simulink model "sf_battery_management"  (R2025b)
settings: Solver=FixedStepAuto  StartTime=0.0  StopTime=inf  FixedStep=0.1  RelTol=1e-3
PreLoadFcn:
  | load('battery_management_data.mat')
values from neighbouring files (symbols this model uses):
  CODEGEN_FLAG = 0    [battery_management_data.mat]
  currentFaultSim = 0    [battery_management_data.mat]
  currentSensorSim = 0    [battery_management_data.mat]
  tempFaultSim = 0    [battery_management_data.mat]
  tempSensorSim = 0    [battery_management_data.mat]
  voltageFaultSim = 0    [battery_management_data.mat]
  voltageSensorSim = 0    [battery_management_data.mat]
(part 2 of 3)

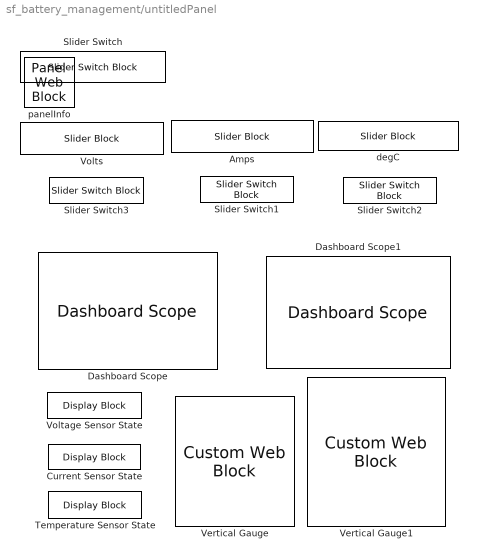
== system sf_battery_management/untitledPanel ==
  Amps : SliderBlock  Tag=HiddenForWebPanel  PanelInfo="{\"height\":32,\"left\":162,\"panelId\":\"panelId-91335c16-9517-4c37-953d-f6a6e757ae52\",\"top\":78,\"type\":\"panelChild\",\"version\":\"2019b\",\"width\":142,\"zIndex\":2000844}"  LabelPosition=Hide  ScaleMax=500  TickInterval=125
  Current Sensor State : DisplayBlock  Tag=HiddenForWebPanel  PanelInfo="{\"height\":25,\"left\":39,\"panelId\":\"panelId-91335c16-9517-4c37-953d-f6a6e757ae52\",\"top\":402,\"type\":\"panelChild\",\"version\":\"2019b\",\"width\":92,\"zIndex\":1500016}"  LabelPosition=Hide  Transparency=1  GridColor=[0.502, 0.502, 0.502]
  Dashboard Scope : DashboardScope  Tag=HiddenForWebPanel  PanelInfo="{\"height\":117,\"left\":29,\"panelId\":\"panelId-91335c16-9517-4c37-953d-f6a6e757ae52\",\"top\":210,\"type\":\"panelChild\",\"version\":\"2019b\",\"width\":179,\"zIndex\":2000856}"  TimeSpan=10  Ymin=100  Ymax=300  LegendPosition=Hide  ScaleAtStop=off  FontColor=[0.0, 0.0, 0.0]
  Dashboard Scope1 : DashboardScope  Tag=HiddenForWebPanel  PanelInfo="{\"height\":112,\"left\":257,\"panelId\":\"panelId-91335c16-9517-4c37-953d-f6a6e757ae52\",\"top\":214,\"type\":\"panelChild\",\"version\":\"2019b\",\"width\":184,\"zIndex\":2000858}"  TimeSpan=10  Ymin=0  Ymax=100  LegendPosition=Hide  ScaleAtStop=off  FontColor=[0.0, 0.0, 0.0]
  Slider Switch : SliderSwitchBlock  Tag=HiddenForWebPanel  PanelInfo="{\"height\":31,\"left\":11,\"panelId\":\"panelId-91335c16-9517-4c37-953d-f6a6e757ae52\",\"top\":9,\"type\":\"panelChild\",\"version\":\"2019b\",\"width\":145,\"zIndex\":2000854}"  LabelPosition=Hide
  Slider Switch1 : SliderSwitchBlock  Tag=HiddenForWebPanel  PanelInfo="{\"height\":26,\"left\":191,\"panelId\":\"panelId-91335c16-9517-4c37-953d-f6a6e757ae52\",\"top\":134,\"type\":\"panelChild\",\"version\":\"2019b\",\"width\":93,\"zIndex\":2000862}"  LabelPosition=Hide
  Slider Switch2 : SliderSwitchBlock  Tag=HiddenForWebPanel  PanelInfo="{\"height\":26,\"left\":334,\"panelId\":\"panelId-91335c16-9517-4c37-953d-f6a6e757ae52\",\"top\":135,\"type\":\"panelChild\",\"version\":\"2019b\",\"width\":93,\"zIndex\":2000864}"  LabelPosition=Hide
  Slider Switch3 : SliderSwitchBlock  Tag=HiddenForWebPanel  PanelInfo="{\"height\":26,\"left\":40,\"panelId\":\"panelId-91335c16-9517-4c37-953d-f6a6e757ae52\",\"top\":135,\"type\":\"panelChild\",\"version\":\"2019b\",\"width\":94,\"zIndex\":2000860}"  LabelPosition=Hide
  Temperature Sensor State : DisplayBlock  Tag=HiddenForWebPanel  PanelInfo="{\"height\":27,\"left\":39,\"panelId\":\"panelId-91335c16-9517-4c37-953d-f6a6e757ae52\",\"top\":449,\"type\":\"panelChild\",\"version\":\"2019b\",\"width\":93,\"zIndex\":1500014}"  LabelPosition=Hide  Transparency=1  GridColor=[0.502, 0.502, 0.502]
  Vertical Gauge : CustomWebBlock  Tag=HiddenForWebPanel  PanelInfo="{\"height\":130,\"left\":166,\"panelId\":\"panelId-91335c16-9517-4c37-953d-f6a6e757ae52\",\"top\":354,\"type\":\"panelChild\",\"version\":\"2019b\",\"width\":119,\"zIndex\":1500008}"  LabelPosition=Hide  ShowInitialText=on  Configuration="{\"components\":[{\"name\":\"LinearScaleComponent\",\"settings\":{\"bounds\":{\"max\":4.5,\"min\":-0.5,\"tickInterval\":1},\"labelColor\":[0,85,255],\"labelFont\":{\"font\":\"Arial\",\"fontSize\":12},\"labelOffset\":0.05,\"labelTransparency\":0,\"needleImage\":{\"size\":[109,53],\"src\":\"data:image\\/png;base64,iVBORw0KGgoAAAANSUhEUgAAAG0AAAA1CAMAAAB8+5X+AAAAAXNSR0IArs4c6QAAAARnQU1BAACxjwv8YQUAAAByUExURQAAAP8AAP8AAP8AAP8AAP8AAP8AAP8AAP8AAP8AAP8AAP8AAP8AAP8AAP8AAP8AAP8AAP8AAP8AAP8AAP8AAP8AAP8AAP8AAP8AAP8AAP8AAP8AAP8AAP8AAP8AAP8AAP8AAP8AAP8AAP8AAP8AAP8AAImxNnoAAAAldFJOUwAEDBAUGBwgJDQ4PFBUWHR4fICTl5ufo6+zt7u\\/w8\\/T1+fz9\\/snRUfzAAAACXBIWXMAABcRAAAXEQHKJvM\\/AAABCUlEQVRYR92Yxw7CQAxEQ++99ySw\\/\\/+LlDyJAAsnew68E9iWRxFDdu0kmDKrJD+hzIpNlb5xqDLj2KBxFIrsyDp0jkGNIXmf1hEoseQyovcnVNgy\\/2ZN8sZsv1iTtDWnJv1fIWtO3Jok7ckHKJQh58EYiRJkXFh8WJOED7t3axJ3Im0hA4S9yLroFBB1Ix8i9ICgIxOU7hDyZPm0JhFX9jXEJGohbSvVQtZTqoVzYU2++TOVqoXVzZp8VHCoK9XC+m+fTfq7KT0p\\/b9J3yXS96T0DJCeb8qzW3ovkd65pPdJ6V1ZOgcoZxzp\\/CadTaVzt3SnoNyXSHdB0j2XdIcn3U9Kd68\\/98pJcgVZGsxjzJl\\/4AAAAABJRU5ErkJggg==\",\"srcOrientation\":\"Right\"},\"needleOffset\":[-0.0013831258644536654,-0.18488023952095808],\"needleSize\":{\"height\":0.07432154605263158,\"width\":0.1941860465116279},\"position\":[0.2313939144736842,0.12056686046511628,0.41540697674418603,0.6739823190789473],\"referencePoint\":\"auto\",\"scaleColorSize\":0.24,\"scaleColors\":[],\"scaleColorsSize\":0.2,\"scaleDirection\":\"BT\",\"tickColor\":[0,0,0],\"tickTransparency\":0.8,\"valueBarColor\":[81,255,0],\"valueBarSize\":0.23,\"valueBarTransparency\":1}},{\"name\":\"BackgroundImageComponent\",\"settings\":{\"image\":{\"size\":[776,978],\"src\":\"data:image\\/png;base64,iVBORw0KGgoAAAANSUhEUgAAAwgAAAPSCAYAAADfoP1eAAAAAXNSR0IArs4c6QAAAARnQU1BAACxjwv8YQUAAAAJcEhZcwAAFxEAABcRAcom8z8AAN6TSURBVHhe7P1ZuB1Xde\\/9\\/y\\/OxXtxLs7FuTgX53ne9+I8cSsJAgSSkNCEA4TWsiEhIaFJSEhHQughELoAobFkg8GAgzEY95ZkNZas3pYty5Z7tVbfd1bf91r\\/Gku15a2t315zzlpzrVVjr+\\/g+TyAvWtWrbn3nDXGqqpZ\\/z\\/Cf1x97Q8uH33NDe8ac+34jzSNHf+1pmvH3zx67LhfFv99X\\/Hf88dcO+7R0deO22CKf3+8+OcNAADgw+hrx5++cB63c3pxbi9MKs ...(+78488 chars)\",\"srcOrientation\":\"vertical\"},\"position\":[0,0,1,1],\"scaleMode\":\"0\"}},{\"name\":\"ForegroundImageComponent\",\"settings\":{\"image\":{\"size\":[0,0],\"src\":\"default\",\"srcOrientation\":\"\"},\"isForeground\":1,\"position\":[0,0,1,1]}}],\"derived\":{\"blockParameters\":{\"ForegroundColor\":[0,0,0],\"Limits\":{\"Max\":4.5,\"Min\":-0.5,\"Ticks\":1},\"ScaleColors\":[],\"ScaleDirection\":\"Clockwise\",\"ScaleMax\":4.5,\"ScaleMin\":-0.5,\"TickInterval\":1,\"fixedAspectRatio\":\"on\"}},\"settings\":{\"BindingType\":\"signal\",\"backgroundColor\":[0,0,0],\"backgroundOffset\":0,\"backgroundOpacity\":1,\"fixedAspectRatio\":\"on\",\"orientation\":\"vertical\",\"showBackgroundColor\":0,\"version\":\"R2025a\"},\"type\":\"LinearGauge\"}"
  Vertical Gauge1 : CustomWebBlock  Tag=HiddenForWebPanel  PanelInfo="{\"height\":149,\"left\":298,\"panelId\":\"panelId-91335c16-9517-4c37-953d-f6a6e757ae52\",\"top\":335,\"type\":\"panelChild\",\"version\":\"2019b\",\"width\":138,\"zIndex\":1500022}"  LabelPosition=Hide  ShowInitialText=on  Configuration="{\"components\":[{\"name\":\"LinearScaleComponent\",\"settings\":{\"bounds\":{\"max\":2.5,\"min\":-2.5,\"tickInterval\":1},\"labelColor\":[0,85,255],\"labelFont\":{\"font\":\"Arial\",\"fontSize\":12},\"labelOffset\":0.05,\"labelTransparency\":0,\"needleImage\":{\"size\":[80,81],\"src\":\"data:image\\/png;base64,iVBORw0KGgoAAAANSUhEUgAAAFAAAABRCAMAAAByk9E6AAAAAXNSR0IArs4c6QAAAARnQU1BAACxjwv8YQUAAADVUExURQAAAEBAgCBggDBQjytVii5SkjJVji1TjDBQjy9RkTBUjzBTjy5SjzBSjy5SjzBSjy5RjzBSjy9SjjBTjy5SjzBSjy9Sjy9Sjy9Tji9SkC9Rjy9Sjy5Sjy9Tjy9SkC9Sjy9Sjy9SkC9Sjy9Sjy9SkC9SjzBSkjBUky9Sjy9TkDBSkTBTkTBUkjFVlDJWlzNYmTRZmzRanDVbnjVcnzZdoTdeozhgpjlhqDpiqjpjqztkrTxmsD5otD9qt0BsukBsu0FuvEFuvUJvv0NwwUNxwkRxw0RyxLvf0MQAAAAodFJOUwAECBAYHCQoMDxAUFRgZHB0gIOLj5ufr7O3v8PLz9fb4+fr7\\/f7\\/v5uSHl1AAAACXBIWXMAABcRAAAXEQHKJvM\\/AAAB+0lEQVRYR63Y2VbCMBAG4Ir7voviioLGfQVRBJFl3v+RnNAUCm3TyWT+u\\/Yk3017JpMJ1mcC2ahzYVIpYVKpRyTXzJNAlOp\\/I3m6ap69oxSAKKlBUTIENfkgQ0YgQK+B5MmKec\\/OGDRkyZOMgyLkJChAToNIft77kEkQoFtH8nDJrHBMGqjJO6WKLDId9CCzQDaZDSJZu3UnbSBAB8nqwYJZS4odZJB5oDOZDzqSFBDg910hOW\\/2WEMDAdpIVvbmzC5LqCCZpINE0gUkkW4gQOsVyd1ZszslrmBIXm1nku5gDskBrSQPRPIlg+SCAD\\/PSG4VjDMKHwzJ8uYU6QOmkn5gCukLIvk0QfqDMGgieRH11QKgIU2rLgLGSSEQyQ+8UBwVxMDR15YBYz+PBKi5y+jH8QdbyMXKhC+YKGR+YEpd9AFTyywf1FxlJ1FiuWD7LeNA5YGW85kDWo97dzCne3AFNVfdtzQjbmCnpvtEa+vpApI6WTpIbIypILnPpoF\\/yKniotljDQXs1q\\/pN6p80InLBx25PJBxI7WBPc2Vls1KYrLBXuOGM3vIAplcFsjm0sHh7OaYOWhJgv0v5PhjtWnQe\\/A3CQrMEeOgyFhyDA65M++RZAQOmshJDKBDMN4ke0aDgpwGRTkNIlfekOI0OH1Z84wwFwSyXBD8AwOyKt7SV8XcAAAAAElFTkSuQmCC\",\"srcOrientation\":\"Right\"},\"needleOffset\":[-0.03305785123966942,-0.28908964558721334],\"needleSize\":{\"height\":0.1281779661016949,\"width\":0.08817401960784314},\"position\":[0.1421875,0.19939630681818182,0.2859552556818182,0.8486842105263158],\"referencePoint\":\"auto\",\"scaleColorSize\":0.24,\"scaleColors\":[],\"scaleColorsSize\":0.2,\"scaleDirection\":\"BT\",\"tickColor\":[0,0,0],\"tickTransparency\":0.9,\"valueBarColor\":[81,255,0],\"valueBarSize\":0.23,\"valueBarTransparency\":0}},{\"name\":\"BackgroundImageComponent\",\"settings\":{\"image\":{\"size\":[852,986],\"src\":\"data:image\\/png;base64,iVBORw0KGgoAAAANSUhEUgAAA1QAAAPaCAYAAACQ2xn1AAAAAXNSR0IArs4c6QAAAARnQU1BAACxjwv8YQUAAAAJcEhZcwAAFxEAABcRAcom8z8AAOWhSURBVHhe7P1rtDVnXed754UvfLGHyYt+0S\\/2EB3DwX1ed8IxQPAGEpIYCMm6E5SD4dwQWg42IRhAzAEldkjWCgpiGyGgtlE5oy0ICO7dqBt9xqPI2Nt2d6tt293SQ3sjjTY+0L3Xs35zrUrmXfldV9X\\/qqo5q2p+rzE+Su5Vp1lVs+b\\/V4erzqNtZjtz5tZvOXn27qOnr9t9yqntnetPn9190da1Ozee3t69beHs7ru3tnfu3\\/\\/\\/H9j\\/\\/59bOLvz54e+sv\\/vew ...(+80792 chars)\",\"srcOrientation\":\"vertical\"},\"position\":[0,0,1,1],\"scaleMode\":\"0\"}},{\"name\":\"ForegroundImageComponent\",\"settings\":{\"image\":{\"size\":[0,0],\"src\":\"default\",\"srcOrientation\":\"\"},\"isForeground\":1,\"position\":[0,0,1,1]}}],\"derived\":{\"blockParameters\":{\"ForegroundColor\":[0,0,0],\"Limits\":{\"Max\":2.5,\"Min\":-2.5,\"Ticks\":1},\"ScaleColors\":[],\"ScaleDirection\":\"Clockwise\",\"ScaleMax\":2.5,\"ScaleMin\":-2.5,\"TickInterval\":1,\"fixedAspectRatio\":\"on\"}},\"settings\":{\"BindingType\":\"signal\",\"backgroundColor\":[0,0,0],\"backgroundOffset\":0,\"backgroundOpacity\":1,\"fixedAspectRatio\":\"on\",\"orientation\":\"vertical\",\"showBackgroundColor\":0,\"version\":\"R2025a\"},\"type\":\"LinearGauge\"}"
  Voltage Sensor State : DisplayBlock  Tag=HiddenForWebPanel  PanelInfo="{\"height\":26,\"left\":38,\"panelId\":\"panelId-91335c16-9517-4c37-953d-f6a6e757ae52\",\"top\":350,\"type\":\"panelChild\",\"version\":\"2019b\",\"width\":94,\"zIndex\":1500018}"  LabelPosition=Hide  Transparency=1  GridColor=[0.502, 0.502, 0.502]
  Volts : SliderBlock  Tag=HiddenForWebPanel  PanelInfo="{\"height\":32,\"left\":11,\"panelId\":\"panelId-91335c16-9517-4c37-953d-f6a6e757ae52\",\"top\":80,\"type\":\"panelChild\",\"version\":\"2019b\",\"width\":143,\"zIndex\":2000842}"  LabelPosition=Hide  ScaleMin=100  ScaleMax=300  TickInterval=100
  degC : SliderBlock  Tag=HiddenForWebPanel  PanelInfo="{\"height\":29,\"left\":309,\"panelId\":\"panelId-91335c16-9517-4c37-953d-f6a6e757ae52\",\"top\":79,\"type\":\"panelChild\",\"version\":\"2019b\",\"width\":140,\"zIndex\":2000846}"  LabelPosition=Hide  ScaleMin=-50  ScaleMax=50  TickInterval=25
  panelInfo : PanelWebBlock  Tag=HiddenForWebPanel  PanelInfo="{\"compacted\":false,\"height\":496,\"isActiveTab\":true,\"labels\":{\"label0480254190\":{\"left\":\"244\",\"settings\":{\"backgroundColor\":\"rgba(0, 0, 0, 0)\",\"bold\":false,\"font\":\"Arial\",\"fontColor\":\"black\",\"fontSize\":0.71,\"italicized\":false,\"underlined\":false},\"text\":\"%\",\"top\":\"252\"},\"label1417532565\":{\"left\":\"170\",\"settings\":{\"backgroundColor\":\"rgba(0, 0, 0, 0)\",\"bold\":true,\"font\":\"Arial\",\"fontColor\":\"black\",\"fontSize\":0.86,\"italicized\":false,\"underlined\":false},\"text\":\"Signal Monitoring\",\"top\":\"172\"},\"label2677336777\":{\"left\":\"164\",\"settings\":{\"backgroundColor\":\"rgba(0, 0, 0, 0)\",\"bold\":true,\"font\":\"Arial\",\"fontColor\":\"black\",\"fontSize\":0.94,\"italicized\":false,\"underlined\":false},\"text\":\"State Monitoring\",\"top\":\"330\"},\"label3169608891\":{\"left\":\"70\",\"settings\":{\"backgroundColor\":\"rgba(0, 0, 0, 0)\",\"bold\":false,\"font\":\"Arial\",\"fontColor\":\"black\",\"fontSize\":0.71,\"italicized\":false,\"underlined\":false},\"text\":\"Voltage read from sensor\",\"top\":\"197\"},\"label4653890763\":{\"left\":\"56\",\"settings\":{\"backgroundColor\":\"rgba(0, 0, 0, 0)\",\"bold\":false,\"font\":\"Arial\",\"fontColor\":\"black\",\"fontSize\":0.71,\"italicized\":false,\"underlined\":false},\"text\":\"Voltage [V]\",\"top\":\"59\"},\"label5267384152\":{\"left\":\"319\",\"settings\":{\"backgroundColor\":\"rgba(0, 0, 0, 0)\",\"bold\":false,\"font\":\"Arial\",\"fontColor\":\"black\",\"fontSize\":0.55,\"italicized\":false,\"underlined\":false},\"text\":\"Send Temperature Error Code\",\"top\":\"123\"},\"label5437745661\":{\"left\":\"37\",\"settings\":{\"backgroundColor\":\"rgba(0, 0, 0, 0)\",\"bold\":false,\"font\":\"Arial\",\"fontColor\":\"black\",\"fontSize\":0.55,\"italicized\":false,\"underlined\":false},\"text\":\"Send Voltage Error Code\",\"top\":\"123\"},\"label6942438338\":{\"left\":\"331\",\"settings\":{\"backgroundColor\":\"rgba(0, 0, 0, 0)\",\"bold\":false,\"font\":\"Arial\",\"fontColor\":\"black\",\"fontSize\":0.71,\"italicized\":false,\"underlined\":false},\"text\":\"Temperature [degC]\",\"top\":\"57\"},\"label7286642277\":{\"left\":\"292\",\"settings\":{\"backgroundColor\":\"rgba(0, 0, 0, 0)\",\"bold\":false,\"font\":\"Arial\",\"fontColor\":\"black\",\"fontSize\":0.71,\"italicized\":false,\"underlined\":false},\"text\":\"SOC estimate from C code\",\"top\":\"199\"},\"label7883531891\":{\"left\":\"17\",\"settings\":{\"backgroundColor\":\"rgba(0, 0, 0, 0)\",\"bold\":false,\"font\":\"Arial\",\"fontColor\":\"black\",\"fontSize\":0.71,\"italicized\":false,\"underlined\":false},\"text\":\"Voltage Sensor Fault State\",\"top\":\"336\"},\"label8120698335\":{\"left\":\"205\",\"settings\":{\"backgroundColor\":\"rgba(0, 0, 0, 0)\",\"bold\":false,\"font\":\"Arial\",\"fontColor\":\"black\",\"fontSize\":0.71,\"italicized\":false,\"underlined\":false},\"text\":\"Current [A]\",\"top\":\"61\"},\"label8170647083\":{\"left\":\"9\",\"settings\":{\"backgroundColor\":\"rgba(0, 0, 0, 0)\",\"bold\":false,\"font\":\"Arial\",\"fontColor\":\"black\",\"fontSize\":0.71,\"italicized\":false,\"underlined\":false},\"text\":\"Volts\",\"top\":\"251\"},\"label8292420699\":{\"left\":\"9\",\"settings\":{\"backgroundColor\":\"rgba(0, 0, 0, 0)\",\"bold\":false,\"font\":\"Arial\",\"fontColor\":\"black\",\"fontSize\":0.71,\"italicized\":false,\"underlined\":false},\"text\":\"Temperature Sensor Fault State\",\"top\":\"436\"},\"label8302910947\":{\"left\":\"186\",\"settings\":{\"backgroundColor\":\"rgba(0, 0, 0, 0)\",\"bold\":true,\"font\":\"Arial\",\"fontColor\":\"black\",\"fontSize\":0.94,\"italicized\":false,\"underlined\":false},\"text\":\"Sensor Input\",\"top\":\"7\"},\"label8970115634\":{\"left\":\"18\",\"settings\":{\"backgroundColor\":\"rgba(0, 0, 0, 0)\",\"bold\":false,\"font\":\"Arial\",\"fontColor\":\"black\",\"fontSize\":0.71,\"italicized\":false,\"underlined\":false},\"text\":\"Current Sensor Fault State\",\"top\":\"387\"},\"label9336161722\":{\"left\":\"184\",\"settings\":{\"backgroundColor\":\"rgba(0, 0, 0, 0)\",\"bold\":false,\"font\":\"Arial\",\"fontColor\":\"black\",\"fontSize\":0.55,\"italicized\":false,\"underlined\":false},\"text\":\"Send Current Error Code\",\"top\":\"122\"}},\"left\":39,\"name\":\"untitledPanel\",\"panelId\":\"panelId-91335c16-9517-4c37-953d-f6a6e757ae52\",\"popoutData\":{\"height\":0,\"left\":0,\"maximized\":false,\"top\":0,\"width\":0},\"popoutMode\":\"component\",\"tabIndex\":0,\"tabbedSetId\":\"tabbedSet7134090722\",\"top\":40,\"type\":\"panel\",\"version\":\"2019b\",\"visible\":true,\"width\":451,\"zIndex\":1500002}"  PanelSnapshot=<binary blob, 61748 chars, not shown>  PanelBackground=data:image/png;base64,iVBORw0KGgoAAAANSUhEUgAAAsQAAANHCAMAAAAG2LtzAAAAAXNSR0IArs4c6QAAAARnQU1BAACxjwv8YQUAAAAJUExURX9/f+v//wAAAKvL7AYAAAADdFJOU///ANfKDUEAAAAJcEhZcwAAFxEAABcRAcom8z8AABAJSURBVHhe7dqhEcQAEAOxfP9NP1l4BTgZCRsu9AMAAAAAAAAAAHzFD16hYC8tYFzBXlrAuIK9tIBxBXtpAeMK9tICxhXspQWMK9hLCxhXsJcWMK5gLy1gXMFeWsC4gr20gHEFe2kB4wr20gLGFeylBYwr2EsLGFewlxYwrmAvLWBcwV5awLiCvbSAcQV7aQHjCvbSAsYV7KUFjCvYSwsYV7CXFjCuYC8tYFzBXlrAuIK9 ...(+5264 chars)
